simulink model "Main_SpeedOptimisedVersionTannenweg"  (R2024b)
settings: Solver=ode15s  StartTime=0.0  StopTime=3600*2  FixedStep=0.1  RelTol=0.001
model workspace (MAT data in the model file):
  Ti = 5
  fa = 0.00071
  fd = 0.03
  ips = 36
  ma = 0.0013
  md = 0.04
  roomarea1 = 20
  s = 15
libraries: fl_lib x1434, nesl_utility x105, SimscapeFluids_lib x35
(part 9 of 22)

== system Main_SpeedOptimisedVersionTannenweg/OG1/Raum3 ==
  Tatm : Inport
  valve command : Inport  Port=2
  Controlled Temperature Source : fl_lib/Thermal/Thermal Sources/Controlled Temperature Source
  Flur3EG : fl_lib/Thermal/Thermal Elements/Convective Heat Transfer  thermal_type=foundation.enum.constant_variable.constant  area=15.87 m^2  heat_tr_coeff=.8 W/m^2/K  min_heat_tr_coeff=1e-3 W/(K*m^2)  T_specify=off  T_priority=High  T=0 K  T_nominal_specify=off  T_nominal_value=1  T_nominal_unit=K  Q_specify=off  Q_priority=High  Q=0 J/s  Q_nominal_specify=off  Q_nominal_value=1  Q_nominal_unit=W
  Flur3OG2 : fl_lib/Thermal/Thermal Elements/Convective Heat Transfer  thermal_type=foundation.enum.constant_variable.constant  area=15.87 m^2  heat_tr_coeff=.8 W/m^2/K  min_heat_tr_coeff=1e-3 W/(K*m^2)  T_specify=off  T_priority=High  T=0 K  T_nominal_specify=off  T_nominal_value=1  T_nominal_unit=K  Q_specify=off  Q_priority=High  Q=0 J/s  Q_nominal_specify=off  Q_nominal_value=1  Q_nominal_unit=W
  Half Flur3EG : fl_lib/Thermal/Thermal Elements/Conductive Heat Transfer  thermal_type=foundation.enum.ConstantVariableTabulated.Constant  wall_geometry=foundation.enum.ConductionWallGeometry.Planar  area=15.87 m^2  thickness=.15 m  d_in=0.05 m  d_out=0.1 m  L=1 m  th_cond_min=10 W/(K*m)  th_cond=.32 W/m/K  th_cond_TLU=[413, 401, 392, 383, 371, 357, 342] W/(K*m)  temp_TLU=[200, 273, 400, 600, 800, 1000, 1200] K  T_specify=off  T_priority=High  T=0 K  T_nominal_specify=off  T_nominal_value=1  T_nominal_unit=K  Q_specify=off  Q_priority=High  Q=0 J/s  Q_nominal_specify=off  Q_nominal_value=1  Q_nominal_unit=W
  Half Flur3OG2 : fl_lib/Thermal/Thermal Elements/Conductive Heat Transfer  thermal_type=foundation.enum.ConstantVariableTabulated.Constant  wall_geometry=foundation.enum.ConductionWallGeometry.Planar  area=15.87 m^2  thickness=.15 m  d_in=0.05 m  d_out=0.1 m  L=1 m  th_cond_min=10 W/(K*m)  th_cond=.32 W/m/K  th_cond_TLU=[413, 401, 392, 383, 371, 357, 342] W/(K*m)  temp_TLU=[200, 273, 400, 600, 800, 1000, 1200] K  T_specify=off  T_priority=High  T=0 K  T_nominal_specify=off  T_nominal_value=1  T_nominal_unit=K  Q_specify=off  Q_priority=High  Q=0 J/s  Q_nominal_specify=off  Q_nominal_value=1  Q_nominal_unit=W
  Half IT-Air1 : fl_lib/Thermal/Thermal Elements/Conductive Heat Transfer  thermal_type=foundation.enum.ConstantVariableTabulated.Constant  wall_geometry=foundation.enum.ConductionWallGeometry.Planar  area=1.8 m^2  thickness=.022 m  d_in=0.05 m  d_out=0.1 m  L=1 m  th_cond_min=10 W/(K*m)  th_cond=.13 W/m/K  th_cond_TLU=[413, 401, 392, 383, 371, 357, 342] W/(K*m)  temp_TLU=[200, 273, 400, 600, 800, 1000, 1200] K  T_specify=off  T_priority=High  T=0 K  T_nominal_specify=off  T_nominal_value=1  T_nominal_unit=K  Q_specify=off  Q_priority=High  Q=0 J/s  Q_nominal_specify=off  Q_nominal_value=1  Q_nominal_unit=W
  Half IT-Air2 : fl_lib/Thermal/Thermal Elements/Conductive Heat Transfer  thermal_type=foundation.enum.ConstantVariableTabulated.Constant  wall_geometry=foundation.enum.ConductionWallGeometry.Planar  area=8.4 m^2  thickness=.022 m  d_in=0.05 m  d_out=0.1 m  L=1 m  th_cond_min=10 W/(K*m)  th_cond=.13 W/m/K  th_cond_TLU=[413, 401, 392, 383, 371, 357, 342] W/(K*m)  temp_TLU=[200, 273, 400, 600, 800, 1000, 1200] K  T_specify=off  T_priority=High  T=0 K  T_nominal_specify=off  T_nominal_value=1  T_nominal_unit=K  Q_specify=off  Q_priority=High  Q=0 J/s  Q_nominal_specify=off  Q_nominal_value=1  Q_nominal_unit=W
  Half IW1-Air : fl_lib/Thermal/Thermal Elements/Conductive Heat Transfer  thermal_type=foundation.enum.ConstantVariableTabulated.Constant  wall_geometry=foundation.enum.ConductionWallGeometry.Planar  area=6.7 m^2  thickness=.16 m  d_in=0.05 m  d_out=0.1 m  L=1 m  th_cond_min=10 W/(K*m)  th_cond=.069 W/m/K  th_cond_TLU=[413, 401, 392, 383, 371, 357, 342] W/(K*m)  temp_TLU=[200, 273, 400, 600, 800, 1000, 1200] K  T_specify=off  T_priority=High  T=0 K  T_nominal_specify=off  T_nominal_value=1  T_nominal_unit=K  Q_specify=off  Q_priority=High  Q=0 J/s  Q_nominal_specify=off  Q_nominal_value=1  Q_nominal_unit=W
  Half IW1-Air1 : fl_lib/Thermal/Thermal Elements/Conductive Heat Transfer  thermal_type=foundation.enum.ConstantVariableTabulated.Constant  wall_geometry=foundation.enum.ConductionWallGeometry.Planar  area=8.5 m^2  thickness=.16 m  d_in=0.05 m  d_out=0.1 m  L=1 m  th_cond_min=10 W/(K*m)  th_cond=.069 W/m/K  th_cond_TLU=[413, 401, 392, 383, 371, 357, 342] W/(K*m)  temp_TLU=[200, 273, 400, 600, 800, 1000, 1200] K  T_specify=off  T_priority=High  T=0 K  T_nominal_specify=off  T_nominal_value=1  T_nominal_unit=K  Q_specify=off  Q_priority=High  Q=0 J/s  Q_nominal_specify=off  Q_nominal_value=1  Q_nominal_unit=W
  Heater : Subsystem
      settings: PortSchema="{\"entries\":[{\"content\":{\"sides\":[{\"content\":{\"connectorIds\":[\"In1\"]},\"type\":\"ConnectorPlacement.EquallySpacedRectSide\",\"uuid\":\"7b4379d5-fe86-4f5f-b347-17463247d5cb\"},{\"content\":{\"connectorIds\":[\"RConn1\"],\"side\":\"RIGHT\"},\"type\":\"ConnectorPlacement.EquallySpacedRectSide\",\"uuid\":\"add3919f-9a79-4726-aacf-5344366c736f\"},{\"content\":{\"connectorIds\":[\"LConn1\"],\"side\":\"TOP\"},\"type\":\"ConnectorPlacement.EquallySpacedRectSide\",\"uuid\":\"2be7b118-9114-410d-904a-4756a3068fbb\"},{\"content\":{\"connectorIds\":[\"RConn2\"],\"side\":\"BOTTOM\"},\"type\":\"ConnectorPlacement.EquallySpacedRectSide\",\"uuid\":\"3477f1e1-5c09-4719-a7a1-17d4fd79a7ad\"}]},\"type\":\"ConnectorPlacement.EquallySpacedConnector\",\"uuid\":\"01d92670-8519-469a-8463-0c3952b88216\"}],\"packageUris\":[\"http://schema.mathworks.com/mf0/Connector/R2020b\"],\"version\":\"1.0\"}"
  IT3 : fl_lib/Thermal/Thermal Elements/Convective Heat Transfer  thermal_type=foundation.enum.constant_variable.constant  area=1.8 m^2  heat_tr_coeff=.8 W/m^2/K  min_heat_tr_coeff=1e-3 W/(K*m^2)  T_specify=off  T_priority=High  T=0 K  T_nominal_specify=off  T_nominal_value=1  T_nominal_unit=K  Q_specify=off  Q_priority=High  Q=0 J/s  Q_nominal_specify=off  Q_nominal_value=1  Q_nominal_unit=W
  IW3-12 : fl_lib/Thermal/Thermal Elements/Convective Heat Transfer  thermal_type=foundation.enum.constant_variable.constant  area=8.4 m^2  heat_tr_coeff=.8 W/m^2/K  min_heat_tr_coeff=1e-3 W/(K*m^2)  T_specify=off  T_priority=High  T=0 K  T_nominal_specify=off  T_nominal_value=1  T_nominal_unit=K  Q_specify=off  Q_priority=High  Q=0 J/s  Q_nominal_specify=off  Q_nominal_value=1  Q_nominal_unit=W
  IW3-2 : fl_lib/Thermal/Thermal Elements/Convective Heat Transfer  thermal_type=foundation.enum.constant_variable.constant  area=6.7 m^2  heat_tr_coeff=.8 W/m^2/K  min_heat_tr_coeff=1e-3 W/(K*m^2)  T_specify=off  T_priority=High  T=0 K  T_nominal_specify=off  T_nominal_value=1  T_nominal_unit=K  Q_specify=off  Q_priority=High  Q=0 J/s  Q_nominal_specify=off  Q_nominal_value=1  Q_nominal_unit=W
  IW3-4 : fl_lib/Thermal/Thermal Elements/Convective Heat Transfer  thermal_type=foundation.enum.constant_variable.constant  area=8.5 m^2  heat_tr_coeff=.8 W/m^2/K  min_heat_tr_coeff=1e-3 W/(K*m^2)  T_specify=off  T_priority=High  T=0 K  T_nominal_specify=off  T_nominal_value=1  T_nominal_unit=K  Q_specify=off  Q_priority=High  Q=0 J/s  Q_nominal_specify=off  Q_nominal_value=1  Q_nominal_unit=W
  Simulink-PS Converter3 : nesl_utility/Simulink-PS Converter  PhysicalDomain=network_engine_domain  SubClassName=ps_input  LeftPortType=input  RightPortType=output  PseudoPeriodic=off  Frequencies=[]  NoiseDistribution=none  NoiseParameters=[]  Unit=degC  AffineConversion=on  FilteringAndDerivatives=zero  SimscapeFilterOrder=1  InputFilterTimeConstant=.001  UdotUserProvided=0
  Temp. Sensor : Subsystem
  Thermal Mass 3-12 : fl_lib/Thermal/Thermal Elements/Thermal Mass  mass_type=foundation.enum.constant_variable.constant  mass=8.4*.15*547 kg  sp_heat=1600 J/kg/K  mass_min=1e-6 kg  num_ports=foundation.enum.numPorts2.one  m_specify=off  m_priority=High  m=1 kg  m_nominal_specify=off  m_nominal_value=1  m_nominal_unit=kg  T_specify=on  T_priority=High  T=Ti degC  T_nominal_specify=off  T_nominal_value=1  T_nominal_unit=K  Q_specify=off  Q_priority=None  Q=0 W  Q_nominal_specify=off  Q_nominal_value=1  Q_nominal_unit=W
  Thermal Mass Air : fl_lib/Thermal/Thermal Elements/Thermal Mass  mass_type=foundation.enum.constant_variable.constant  mass=48.7 kg  sp_heat=1005 J/kg/K  mass_min=1e-6 kg  num_ports=foundation.enum.numPorts2.one  m_specify=off  m_priority=High  m=1 kg  m_nominal_specify=off  m_nominal_value=1  m_nominal_unit=kg  T_specify=on  T_priority=High  T=Ti degC  T_nominal_specify=off  T_nominal_value=1  T_nominal_unit=K  Q_specify=off  Q_priority=None  Q=0 W  Q_nominal_specify=off  Q_nominal_value=1  Q_nominal_unit=W
  Thermal Mass Door3 : fl_lib/Thermal/Thermal Elements/Thermal Mass  mass_type=foundation.enum.constant_variable.constant  mass=36 kg  sp_heat=1600 J/kg/K  mass_min=1e-6 kg  num_ports=foundation.enum.numPorts2.one  m_specify=off  m_priority=High  m=1 kg  m_nominal_specify=off  m_nominal_value=1  m_nominal_unit=kg  T_specify=on  T_priority=High  T=Ti degC  T_nominal_specify=off  T_nominal_value=1  T_nominal_unit=K  Q_specify=off  Q_priority=None  Q=0 W  Q_nominal_specify=off  Q_nominal_value=1  Q_nominal_unit=W
  Thermal Mass Flur3EG : fl_lib/Thermal/Thermal Elements/Thermal Mass  mass_type=foundation.enum.constant_variable.constant  mass=4473 kg  sp_heat=889 J/kg/K  mass_min=1e-6 kg  num_ports=foundation.enum.numPorts2.one  m_specify=off  m_priority=High  m=1 kg  m_nominal_specify=off  m_nominal_value=1  m_nominal_unit=kg  T_specify=on  T_priority=High  T=Ti degC  T_nominal_specify=off  T_nominal_value=1  T_nominal_unit=K  Q_specify=off  Q_priority=None  Q=0 W  Q_nominal_specify=off  Q_nominal_value=1  Q_nominal_unit=W
  Thermal Mass Flur3OG2 : fl_lib/Thermal/Thermal Elements/Thermal Mass  mass_type=foundation.enum.constant_variable.constant  mass=4473 kg  sp_heat=889 J/kg/K  mass_min=1e-6 kg  num_ports=foundation.enum.numPorts2.one  m_specify=off  m_priority=High  m=1 kg  m_nominal_specify=off  m_nominal_value=1  m_nominal_unit=kg  T_specify=on  T_priority=High  T=Ti degC  T_nominal_specify=off  T_nominal_value=1  T_nominal_unit=K  Q_specify=off  Q_priority=None  Q=0 W  Q_nominal_specify=off  Q_nominal_value=1  Q_nominal_unit=W
  Thermal Mass IW3-2 : fl_lib/Thermal/Thermal Elements/Thermal Mass  mass_type=foundation.enum.constant_variable.constant  mass=6.7*.15*547 kg  sp_heat=1600 J/kg/K  mass_min=1e-6 kg  num_ports=foundation.enum.numPorts2.one  m_specify=off  m_priority=High  m=1 kg  m_nominal_specify=off  m_nominal_value=1  m_nominal_unit=kg  T_specify=on  T_priority=High  T=Ti degC  T_nominal_specify=off  T_nominal_value=1  T_nominal_unit=K  Q_specify=off  Q_priority=None  Q=0 W  Q_nominal_specify=off  Q_nominal_value=1  Q_nominal_unit=W
  Thermal Mass IW3-4 : fl_lib/Thermal/Thermal Elements/Thermal Mass  mass_type=foundation.enum.constant_variable.constant  mass=8.5*.15*547 kg  sp_heat=1600 J/kg/K  mass_min=1e-6 kg  num_ports=foundation.enum.numPorts2.one  m_specify=off  m_priority=High  m=1 kg  m_nominal_specify=off  m_nominal_value=1  m_nominal_unit=kg  T_specify=on  T_priority=High  T=Ti degC  T_nominal_specify=off  T_nominal_value=1  T_nominal_unit=K  Q_specify=off  Q_priority=None  Q=0 W  Q_nominal_specify=off  Q_nominal_value=1  Q_nominal_unit=W
  Thermal Reference1 : fl_lib/Thermal/Thermal Elements/Thermal Reference
  X-Atm : Subsystem
  Hot Water In1 : PMIOPort  Side=Left
  Y-Flur3OG2 : PMIOPort  Port=2  Side=Left
  Y-Flur3EG : PMIOPort  Port=3  Side=Left
  3-12 : PMIOPort  Port=4  Side=Left
  Door3 : PMIOPort  Port=5  Side=Left
  3-2 : PMIOPort  Port=6  Side=Right
  3-4 : PMIOPort  Port=7  Side=Right
  Hot Water Out1 : PMIOPort  Port=8  Side=Right
  Troom : Outport
  wires:
  Tatm/1 -> Simulink-PS Converter3/1
  Temp. Sensor/1(T) -> Troom/1
  valve command/1 -> Heater/1(valve command)
  connections:
  Flur3OG2/RConn1 -- Half Flur3OG2/LConn1
  Half Flur3OG2/RConn1 -- Y-Flur3OG2/RConn1 -- Thermal Mass Flur3OG2/LConn1
  IT3/RConn1 -- Half IT-Air1/LConn1
  Half IT-Air1/RConn1 -- Door3/RConn1 -- Thermal Mass Door3/LConn1
  IW3-12/RConn1 -- Half IT-Air2/LConn1
  3-12/RConn1 -- Thermal Mass 3-12/LConn1 -- Half IT-Air2/RConn1
  IW3-4/RConn1 -- Half IW1-Air1/LConn1
  3-4/RConn1 -- Half IW1-Air1/RConn1 -- Thermal Mass IW3-4/LConn1
  Heater/RConn2 -- Hot Water Out1/RConn1
  Hot Water In1/RConn1 -- Heater/LConn1
  X-Atm/RConn1 -- Controlled Temperature Source/LConn1
  Flur3EG/LConn1 -- Flur3OG2/LConn1 -- IW3-4/LConn1 -- Heater/RConn1 -- Thermal Mass Air/LConn1 -- X-Atm/LConn1 -- Temp. Sensor/LConn1 -- IW3-2/LConn1 -- IW3-12/LConn1 -- IT3/LConn1
  Controlled Temperature Source/RConn1 -- Simulink-PS Converter3/RConn1
  Thermal Reference1/LConn1 -- Controlled Temperature Source/RConn2
  Half IW1-Air/RConn1 -- Thermal Mass IW3-2/LConn1 -- 3-2/RConn1
  IW3-2/RConn1 -- Half IW1-Air/LConn1
  Half Flur3EG/RConn1 -- Thermal Mass Flur3EG/LConn1 -- Y-Flur3EG/RConn1
  Flur3EG/RConn1 -- Half Flur3EG/LConn1

== system Main_SpeedOptimisedVersionTannenweg/OG1/Raum4 ==
  valve command : Inport
  Tatm : Inport  Port=2
  Air-InnerDoor Convection1 : fl_lib/Thermal/Thermal Elements/Convective Heat Transfer  thermal_type=foundation.enum.constant_variable.constant  area=1.5 m^2  heat_tr_coeff=.8 W/m^2/K  min_heat_tr_coeff=1e-3 W/(K*m^2)  T_specify=off  T_priority=High  T=0 K  T_nominal_specify=off  T_nominal_value=1  T_nominal_unit=K  Q_specify=off  Q_priority=High  Q=0 J/s  Q_nominal_specify=off  Q_nominal_value=1  Q_nominal_unit=W
  Air-InnerWall IW4-1 : fl_lib/Thermal/Thermal Elements/Convective Heat Transfer  thermal_type=foundation.enum.constant_variable.constant  area=7.2 m^2  heat_tr_coeff=.8 W/m^2/K  min_heat_tr_coeff=1e-3 W/(K*m^2)  T_specify=off  T_priority=High  T=0 K  T_nominal_specify=off  T_nominal_value=1  T_nominal_unit=K  Q_specify=off  Q_priority=High  Q=0 J/s  Q_nominal_specify=off  Q_nominal_value=1  Q_nominal_unit=W
  Air-InnerWall IW4-2 : fl_lib/Thermal/Thermal Elements/Convective Heat Transfer  thermal_type=foundation.enum.constant_variable.constant  area=5.2 m^2  heat_tr_coeff=.8 W/m^2/K  min_heat_tr_coeff=1e-3 W/(K*m^2)  T_specify=off  T_priority=High  T=0 K  T_nominal_specify=off  T_nominal_value=1  T_nominal_unit=K  Q_specify=off  Q_priority=High  Q=0 J/s  Q_nominal_specify=off  Q_nominal_value=1  Q_nominal_unit=W
  Air-InnerWall IW4-3 : fl_lib/Thermal/Thermal Elements/Convective Heat Transfer  thermal_type=foundation.enum.constant_variable.constant  area=6.7 m^2  heat_tr_coeff=.8 W/m^2/K  min_heat_tr_coeff=1e-3 W/(K*m^2)  T_specify=off  T_priority=High  T=0 K  T_nominal_specify=off  T_nominal_value=1  T_nominal_unit=K  Q_specify=off  Q_priority=High  Q=0 J/s  Q_nominal_specify=off  Q_nominal_value=1  Q_nominal_unit=W
  Controlled Temperature Source : fl_lib/Thermal/Thermal Sources/Controlled Temperature Source
  Flur4EG : fl_lib/Thermal/Thermal Elements/Convective Heat Transfer  thermal_type=foundation.enum.constant_variable.constant  area=4.53 m^2  heat_tr_coeff=.8 W/m^2/K  min_heat_tr_coeff=1e-3 W/(K*m^2)  T_specify=off  T_priority=High  T=0 K  T_nominal_specify=off  T_nominal_value=1  T_nominal_unit=K  Q_specify=off  Q_priority=High  Q=0 J/s  Q_nominal_specify=off  Q_nominal_value=1  Q_nominal_unit=W
  Flur4OG2 : fl_lib/Thermal/Thermal Elements/Convective Heat Transfer  thermal_type=foundation.enum.constant_variable.constant  area=4.53 m^2  heat_tr_coeff=.8 W/m^2/K  min_heat_tr_coeff=1e-3 W/(K*m^2)  T_specify=off  T_priority=High  T=0 K  T_nominal_specify=off  T_nominal_value=1  T_nominal_unit=K  Q_specify=off  Q_priority=High  Q=0 J/s  Q_nominal_specify=off  Q_nominal_value=1  Q_nominal_unit=W
  Half Flur4EG : fl_lib/Thermal/Thermal Elements/Conductive Heat Transfer  thermal_type=foundation.enum.ConstantVariableTabulated.Constant  wall_geometry=foundation.enum.ConductionWallGeometry.Planar  area=4.53 m^2  thickness=.15 m  d_in=0.05 m  d_out=0.1 m  L=1 m  th_cond_min=10 W/(K*m)  th_cond=.32 W/m/K  th_cond_TLU=[413, 401, 392, 383, 371, 357, 342] W/(K*m)  temp_TLU=[200, 273, 400, 600, 800, 1000, 1200] K  T_specify=off  T_priority=High  T=0 K  T_nominal_specify=off  T_nominal_value=1  T_nominal_unit=K  Q_specify=off  Q_priority=High  Q=0 J/s  Q_nominal_specify=off  Q_nominal_value=1  Q_nominal_unit=W
  Half Flur4OG2 : fl_lib/Thermal/Thermal Elements/Conductive Heat Transfer  thermal_type=foundation.enum.ConstantVariableTabulated.Constant  wall_geometry=foundation.enum.ConductionWallGeometry.Planar  area=4.53 m^2  thickness=.15 m  d_in=0.05 m  d_out=0.1 m  L=1 m  th_cond_min=10 W/(K*m)  th_cond=.32 W/m/K  th_cond_TLU=[413, 401, 392, 383, 371, 357, 342] W/(K*m)  temp_TLU=[200, 273, 400, 600, 800, 1000, 1200] K  T_specify=off  T_priority=High  T=0 K  T_nominal_specify=off  T_nominal_value=1  T_nominal_unit=K  Q_specify=off  Q_priority=High  Q=0 J/s  Q_nominal_specify=off  Q_nominal_value=1  Q_nominal_unit=W
  Half Wall-Air Conduction1 : fl_lib/Thermal/Thermal Elements/Conductive Heat Transfer  thermal_type=foundation.enum.ConstantVariableTabulated.Constant  wall_geometry=foundation.enum.ConductionWallGeometry.Planar  area=7.2 m^2  thickness=.16 m  d_in=0.05 m  d_out=0.1 m  L=1 m  th_cond_min=10 W/(K*m)  th_cond=.069 W/m/K  th_cond_TLU=[413, 401, 392, 383, 371, 357, 342] W/(K*m)  temp_TLU=[200, 273, 400, 600, 800, 1000, 1200] K  T_specify=off  T_priority=High  T=0 K  T_nominal_specify=off  T_nominal_value=1  T_nominal_unit=K  Q_specify=off  Q_priority=High  Q=0 J/s  Q_nominal_specify=off  Q_nominal_value=1  Q_nominal_unit=W
  Half Wall-Air Conduction2 : fl_lib/Thermal/Thermal Elements/Conductive Heat Transfer  thermal_type=foundation.enum.ConstantVariableTabulated.Constant  wall_geometry=foundation.enum.ConductionWallGeometry.Planar  area=5.2 m^2  thickness=.16 m  d_in=0.05 m  d_out=0.1 m  L=1 m  th_cond_min=10 W/(K*m)  th_cond=.069 W/m/K  th_cond_TLU=[413, 401, 392, 383, 371, 357, 342] W/(K*m)  temp_TLU=[200, 273, 400, 600, 800, 1000, 1200] K  T_specify=off  T_priority=High  T=0 K  T_nominal_specify=off  T_nominal_value=1  T_nominal_unit=K  Q_specify=off  Q_priority=High  Q=0 J/s  Q_nominal_specify=off  Q_nominal_value=1  Q_nominal_unit=W
  Half Wall-Air Conduction3 : fl_lib/Thermal/Thermal Elements/Conductive Heat Transfer  thermal_type=foundation.enum.ConstantVariableTabulated.Constant  wall_geometry=foundation.enum.ConductionWallGeometry.Planar  area=6.7 m^2  thickness=.16 m  d_in=0.05 m  d_out=0.1 m  L=1 m  th_cond_min=10 W/(K*m)  th_cond=.069 W/m/K  th_cond_TLU=[413, 401, 392, 383, 371, 357, 342] W/(K*m)  temp_TLU=[200, 273, 400, 600, 800, 1000, 1200] K  T_specify=off  T_priority=High  T=0 K  T_nominal_specify=off  T_nominal_value=1  T_nominal_unit=K  Q_specify=off  Q_priority=High  Q=0 J/s  Q_nominal_specify=off  Q_nominal_value=1  Q_nominal_unit=W
  Half Window-Air Conduction1 : fl_lib/Thermal/Thermal Elements/Conductive Heat Transfer  thermal_type=foundation.enum.ConstantVariableTabulated.Constant  wall_geometry=foundation.enum.ConductionWallGeometry.Planar  area=1.5 m^2  thickness=.022 m  d_in=0.05 m  d_out=0.1 m  L=1 m  th_cond_min=10 W/(K*m)  th_cond=.13 W/m/K  th_cond_TLU=[413, 401, 392, 383, 371, 357, 342] W/(K*m)  temp_TLU=[200, 273, 400, 600, 800, 1000, 1200] K  T_specify=off  T_priority=High  T=0 K  T_nominal_specify=off  T_nominal_value=1  T_nominal_unit=K  Q_specify=off  Q_priority=High  Q=0 J/s  Q_nominal_specify=off  Q_nominal_value=1  Q_nominal_unit=W
  Heater : Subsystem
      settings: PortSchema="{\"entries\":[{\"content\":{\"sides\":[{\"content\":{\"connectorIds\":[\"In1\"]},\"type\":\"ConnectorPlacement.EquallySpacedRectSide\",\"uuid\":\"7b4379d5-fe86-4f5f-b347-17463247d5cb\"},{\"content\":{\"connectorIds\":[\"RConn1\"],\"side\":\"RIGHT\"},\"type\":\"ConnectorPlacement.EquallySpacedRectSide\",\"uuid\":\"add3919f-9a79-4726-aacf-5344366c736f\"},{\"content\":{\"connectorIds\":[\"LConn1\"],\"side\":\"TOP\"},\"type\":\"ConnectorPlacement.EquallySpacedRectSide\",\"uuid\":\"2be7b118-9114-410d-904a-4756a3068fbb\"},{\"content\":{\"connectorIds\":[\"RConn2\"],\"side\":\"BOTTOM\"},\"type\":\"ConnectorPlacement.EquallySpacedRectSide\",\"uuid\":\"3477f1e1-5c09-4719-a7a1-17d4fd79a7ad\"}]},\"type\":\"ConnectorPlacement.EquallySpacedConnector\",\"uuid\":\"01d92670-8519-469a-8463-0c3952b88216\"}],\"packageUris\":[\"http://schema.mathworks.com/mf0/Connector/R2020b\"],\"version\":\"1.0\"}"
  Simulink-PS Converter3 : nesl_utility/Simulink-PS Converter  PhysicalDomain=network_engine_domain  SubClassName=ps_input  LeftPortType=input  RightPortType=output  PseudoPeriodic=off  Frequencies=[]  NoiseDistribution=none  NoiseParameters=[]  Unit=degC  AffineConversion=on  FilteringAndDerivatives=zero  SimscapeFilterOrder=1  InputFilterTimeConstant=.001  UdotUserProvided=0
  Temp. Sensor : Subsystem
  Thermal Mass 4-1 : fl_lib/Thermal/Thermal Elements/Thermal Mass  mass_type=foundation.enum.constant_variable.constant  mass=7.2*.15*547 kg  sp_heat=876 J/kg/K  mass_min=1e-6 kg  num_ports=foundation.enum.numPorts2.one  m_specify=off  m_priority=High  m=1 kg  m_nominal_specify=off  m_nominal_value=1  m_nominal_unit=kg  T_specify=on  T_priority=High  T=Ti degC  T_nominal_specify=off  T_nominal_value=1  T_nominal_unit=K  Q_specify=off  Q_priority=None  Q=0 W  Q_nominal_specify=off  Q_nominal_value=1  Q_nominal_unit=W
  Thermal Mass 4-2 : fl_lib/Thermal/Thermal Elements/Thermal Mass  mass_type=foundation.enum.constant_variable.constant  mass=5.2*.15*547 kg  sp_heat=876 J/kg/K  mass_min=1e-6 kg  num_ports=foundation.enum.numPorts2.one  m_specify=off  m_priority=High  m=1 kg  m_nominal_specify=off  m_nominal_value=1  m_nominal_unit=kg  T_specify=on  T_priority=High  T=Ti degC  T_nominal_specify=off  T_nominal_value=1  T_nominal_unit=K  Q_specify=off  Q_priority=None  Q=0 W  Q_nominal_specify=off  Q_nominal_value=1  Q_nominal_unit=W
  Thermal Mass 4-3 : fl_lib/Thermal/Thermal Elements/Thermal Mass  mass_type=foundation.enum.constant_variable.constant  mass=6.7*.15*547 kg  sp_heat=876 J/kg/K  mass_min=1e-6 kg  num_ports=foundation.enum.numPorts2.one  m_specify=off  m_priority=High  m=1 kg  m_nominal_specify=off  m_nominal_value=1  m_nominal_unit=kg  T_specify=on  T_priority=High  T=Ti degC  T_nominal_specify=off  T_nominal_value=1  T_nominal_unit=K  Q_specify=off  Q_priority=None  Q=0 W  Q_nominal_specify=off  Q_nominal_value=1  Q_nominal_unit=W
  Thermal Mass Air : fl_lib/Thermal/Thermal Elements/Thermal Mass  mass_type=foundation.enum.constant_variable.constant  mass=13.9 kg  sp_heat=1005 J/kg/K  mass_min=1e-6 kg  num_ports=foundation.enum.numPorts2.one  m_specify=off  m_priority=High  m=1 kg  m_nominal_specify=off  m_nominal_value=1  m_nominal_unit=kg  T_specify=on  T_priority=High  T=Ti degC  T_nominal_specify=off  T_nominal_value=1  T_nominal_unit=K  Q_specify=off  Q_priority=None  Q=0 W  Q_nominal_specify=off  Q_nominal_value=1  Q_nominal_unit=W
  Thermal Mass Flur4EG : fl_lib/Thermal/Thermal Elements/Thermal Mass  mass_type=foundation.enum.constant_variable.constant  mass=1277 kg  sp_heat=889 J/kg/K  mass_min=1e-6 kg  num_ports=foundation.enum.numPorts2.one  m_specify=off  m_priority=High  m=1 kg  m_nominal_specify=off  m_nominal_value=1  m_nominal_unit=kg  T_specify=on  T_priority=High  T=Ti degC  T_nominal_specify=off  T_nominal_value=1  T_nominal_unit=K  Q_specify=off  Q_priority=None  Q=0 W  Q_nominal_specify=off  Q_nominal_value=1  Q_nominal_unit=W
  Thermal Mass Flur4OG2 : fl_lib/Thermal/Thermal Elements/Thermal Mass  mass_type=foundation.enum.constant_variable.constant  mass=1277 kg  sp_heat=889 J/kg/K  mass_min=1e-6 kg  num_ports=foundation.enum.numPorts2.one  m_specify=off  m_priority=High  m=1 kg  m_nominal_specify=off  m_nominal_value=1  m_nominal_unit=kg  T_specify=on  T_priority=High  T=Ti degC  T_nominal_specify=off  T_nominal_value=1  T_nominal_unit=K  Q_specify=off  Q_priority=None  Q=0 W  Q_nominal_specify=off  Q_nominal_value=1  Q_nominal_unit=W
  Thermal Mass InnerDoor : fl_lib/Thermal/Thermal Elements/Thermal Mass  mass_type=foundation.enum.constant_variable.constant  mass=30 kg  sp_heat=1600 J/kg/K  mass_min=1e-6 kg  num_ports=foundation.enum.numPorts2.one  m_specify=off  m_priority=High  m=1 kg  m_nominal_specify=off  m_nominal_value=1  m_nominal_unit=kg  T_specify=on  T_priority=High  T=Ti degC  T_nominal_specify=off  T_nominal_value=1  T_nominal_unit=K  Q_specify=off  Q_priority=None  Q=0 W  Q_nominal_specify=off  Q_nominal_value=1  Q_nominal_unit=W
  Thermal Reference1 : fl_lib/Thermal/Thermal Elements/Thermal Reference
  X-Atm : Subsystem
  Hot Water In1 : PMIOPort  Side=Left
  4-3 : PMIOPort  Port=2  Side=Left
  Door4 : PMIOPort  Port=3  Side=Left
  4-2 : PMIOPort  Port=4  Side=Left
  4-1 : PMIOPort  Port=5  Side=Left
  Y-Flur4OG2 : PMIOPort  Port=6  Side=Right
  Y-Flur4EG : PMIOPort  Port=7  Side=Right
  Hot Water Out1 : PMIOPort  Port=8  Side=Right
  Troom : Outport
  wires:
  Tatm/1 -> Simulink-PS Converter3/1
  Temp. Sensor/1(T) -> Troom/1
  valve command/1 -> Heater/1(valve command)
  connections:
  Flur4OG2/RConn1 -- Half Flur4OG2/LConn1
  Half Flur4OG2/RConn1 -- Y-Flur4OG2/RConn1 -- Thermal Mass Flur4OG2/LConn1
  Air-InnerWall IW4-3/RConn1 -- Half Wall-Air Conduction3/LConn1
  Air-InnerWall IW4-2/RConn1 -- Half Wall-Air Conduction2/LConn1
  Air-InnerWall IW4-1/RConn1 -- Half Wall-Air Conduction1/LConn1
  Air-InnerDoor Convection1/RConn1 -- Half Window-Air Conduction1/LConn1
  Thermal Mass 4-3/LConn1 -- 4-3/RConn1 -- Half Wall-Air Conduction3/RConn1
  Door4/RConn1 -- Half Window-Air Conduction1/RConn1 -- Thermal Mass InnerDoor/LConn1
  4-1/RConn1 -- Half Wall-Air Conduction1/RConn1 -- Thermal Mass 4-1/LConn1
  Half Wall-Air Conduction2/RConn1 -- 4-2/RConn1 -- Thermal Mass 4-2/LConn1
  Heater/RConn2 -- Hot Water Out1/RConn1
  Hot Water In1/RConn1 -- Heater/LConn1
  X-Atm/RConn1 -- Controlled Temperature Source/LConn1
  Controlled Temperature Source/RConn1 -- Simulink-PS Converter3/RConn1
  Thermal Reference1/LConn1 -- Controlled Temperature Source/RConn2
  Half Flur4EG/RConn1 -- Thermal Mass Flur4EG/LConn1 -- Y-Flur4EG/RConn1
  Flur4EG/RConn1 -- Half Flur4EG/LConn1
  Flur4EG/LConn1 -- Air-InnerWall IW4-3/LConn1 -- Air-InnerWall IW4-2/LConn1 -- Air-InnerWall IW4-1/LConn1 -- Heater/RConn1 -- Thermal Mass Air/LConn1 -- X-Atm/LConn1 -- Temp. Sensor/LConn1 -- Air-InnerDoor Convection1/LConn1 -- Flur4OG2/LConn1

== system Main_SpeedOptimisedVersionTannenweg/OG1/Raum5 ==
  Tatm : Inport
  valve command : Inport  Port=2
  Air-InnerDoor Convection1 : fl_lib/Thermal/Thermal Elements/Convective Heat Transfer  thermal_type=foundation.enum.constant_variable.constant  area=1.8 m^2  heat_tr_coeff=.8 W/m^2/K  min_heat_tr_coeff=1e-3 W/(K*m^2)  T_specify=off  T_priority=High  T=0 K  T_nominal_specify=off  T_nominal_value=1  T_nominal_unit=K  Q_specify=off  Q_priority=High  Q=0 J/s  Q_nominal_specify=off  Q_nominal_value=1  Q_nominal_unit=W
  Air-InnerWall 5-9 : fl_lib/Thermal/Thermal Elements/Convective Heat Transfer  thermal_type=foundation.enum.constant_variable.constant  area=9.3 m^2  heat_tr_coeff=.8 W/m^2/K  min_heat_tr_coeff=1e-3 W/(K*m^2)  T_specify=off  T_priority=High  T=0 K  T_nominal_specify=off  T_nominal_value=1  T_nominal_unit=K  Q_specify=off  Q_priority=High  Q=0 J/s  Q_nominal_specify=off  Q_nominal_value=1  Q_nominal_unit=W
  Controlled Temperature Source : fl_lib/Thermal/Thermal Sources/Controlled Temperature Source
  Flur5EG : fl_lib/Thermal/Thermal Elements/Convective Heat Transfer  thermal_type=foundation.enum.constant_variable.constant  area=13.58 m^2  heat_tr_coeff=.8 W/m^2/K  min_heat_tr_coeff=1e-3 W/(K*m^2)  T_specify=off  T_priority=High  T=0 K  T_nominal_specify=off  T_nominal_value=1  T_nominal_unit=K  Q_specify=off  Q_priority=High  Q=0 J/s  Q_nominal_specify=off  Q_nominal_value=1  Q_nominal_unit=W
  Flur5OG2 : fl_lib/Thermal/Thermal Elements/Convective Heat Transfer  thermal_type=foundation.enum.constant_variable.constant  area=13.58 m^2  heat_tr_coeff=.8 W/m^2/K  min_heat_tr_coeff=1e-3 W/(K*m^2)  T_specify=off  T_priority=High  T=0 K  T_nominal_specify=off  T_nominal_value=1  T_nominal_unit=K  Q_specify=off  Q_priority=High  Q=0 J/s  Q_nominal_specify=off  Q_nominal_value=1  Q_nominal_unit=W
  Half Flur5EG : fl_lib/Thermal/Thermal Elements/Conductive Heat Transfer  thermal_type=foundation.enum.ConstantVariableTabulated.Constant  wall_geometry=foundation.enum.ConductionWallGeometry.Planar  area=13.58 m^2  thickness=.15 m  d_in=0.05 m  d_out=0.1 m  L=1 m  th_cond_min=10 W/(K*m)  th_cond=.32 W/m/K  th_cond_TLU=[413, 401, 392, 383, 371, 357, 342] W/(K*m)  temp_TLU=[200, 273, 400, 600, 800, 1000, 1200] K  T_specify=off  T_priority=High  T=0 K  T_nominal_specify=off  T_nominal_value=1  T_nominal_unit=K  Q_specify=off  Q_priority=High  Q=0 J/s  Q_nominal_specify=off  Q_nominal_value=1  Q_nominal_unit=W
  Half Flur5OG2 : fl_lib/Thermal/Thermal Elements/Conductive Heat Transfer  thermal_type=foundation.enum.ConstantVariableTabulated.Constant  wall_geometry=foundation.enum.ConductionWallGeometry.Planar  area=13.58 m^2  thickness=.15 m  d_in=0.05 m  d_out=0.1 m  L=1 m  th_cond_min=10 W/(K*m)  th_cond=.32 W/m/K  th_cond_TLU=[413, 401, 392, 383, 371, 357, 342] W/(K*m)  temp_TLU=[200, 273, 400, 600, 800, 1000, 1200] K  T_specify=off  T_priority=High  T=0 K  T_nominal_specify=off  T_nominal_value=1  T_nominal_unit=K  Q_specify=off  Q_priority=High  Q=0 J/s  Q_nominal_specify=off  Q_nominal_value=1  Q_nominal_unit=W
  Half Wall-Air Conduction1 : fl_lib/Thermal/Thermal Elements/Conductive Heat Transfer  thermal_type=foundation.enum.ConstantVariableTabulated.Constant  wall_geometry=foundation.enum.ConductionWallGeometry.Planar  area=9.3 m^2  thickness=.16 m  d_in=0.05 m  d_out=0.1 m  L=1 m  th_cond_min=10 W/(K*m)  th_cond=.069 W/m/K  th_cond_TLU=[413, 401, 392, 383, 371, 357, 342] W/(K*m)  temp_TLU=[200, 273, 400, 600, 800, 1000, 1200] K  T_specify=off  T_priority=High  T=0 K  T_nominal_specify=off  T_nominal_value=1  T_nominal_unit=K  Q_specify=off  Q_priority=High  Q=0 J/s  Q_nominal_specify=off  Q_nominal_value=1  Q_nominal_unit=W
  Half Wall-Air Conduction2 : fl_lib/Thermal/Thermal Elements/Conductive Heat Transfer  thermal_type=foundation.enum.ConstantVariableTabulated.Constant  wall_geometry=foundation.enum.ConductionWallGeometry.Planar  area=2.5 m^2  thickness=.16 m  d_in=0.05 m  d_out=0.1 m  L=1 m  th_cond_min=10 W/(K*m)  th_cond=.069 W/m/K  th_cond_TLU=[413, 401, 392, 383, 371, 357, 342] W/(K*m)  temp_TLU=[200, 273, 400, 600, 800, 1000, 1200] K  T_specify=off  T_priority=High  T=0 K  T_nominal_specify=off  T_nominal_value=1  T_nominal_unit=K  Q_specify=off  Q_priority=High  Q=0 J/s  Q_nominal_specify=off  Q_nominal_value=1  Q_nominal_unit=W
  Half Wall-Air Conduction3 : fl_lib/Thermal/Thermal Elements/Conductive Heat Transfer  thermal_type=foundation.enum.ConstantVariableTabulated.Constant  wall_geometry=foundation.enum.ConductionWallGeometry.Planar  area=9.3 m^2  thickness=.16 m  d_in=0.05 m  d_out=0.1 m  L=1 m  th_cond_min=10 W/(K*m)  th_cond=.069 W/m/K  th_cond_TLU=[413, 401, 392, 383, 371, 357, 342] W/(K*m)  temp_TLU=[200, 273, 400, 600, 800, 1000, 1200] K  T_specify=off  T_priority=High  T=0 K  T_nominal_specify=off  T_nominal_value=1  T_nominal_unit=K  Q_specify=off  Q_priority=High  Q=0 J/s  Q_nominal_specify=off  Q_nominal_value=1  Q_nominal_unit=W
  Half Window-Air Conduction1 : fl_lib/Thermal/Thermal Elements/Conductive Heat Transfer  thermal_type=foundation.enum.ConstantVariableTabulated.Constant  wall_geometry=foundation.enum.ConductionWallGeometry.Planar  area=1.8 m^2  thickness=.022 m  d_in=0.05 m  d_out=0.1 m  L=1 m  th_cond_min=10 W/(K*m)  th_cond=.13 W/m/K  th_cond_TLU=[413, 401, 392, 383, 371, 357, 342] W/(K*m)  temp_TLU=[200, 273, 400, 600, 800, 1000, 1200] K  T_specify=off  T_priority=High  T=0 K  T_nominal_specify=off  T_nominal_value=1  T_nominal_unit=K  Q_specify=off  Q_priority=High  Q=0 J/s  Q_nominal_specify=off  Q_nominal_value=1  Q_nominal_unit=W
  Heater : Subsystem
      settings: PortSchema="{\"entries\":[{\"content\":{\"sides\":[{\"content\":{\"connectorIds\":[\"In1\"]},\"type\":\"ConnectorPlacement.EquallySpacedRectSide\",\"uuid\":\"7b4379d5-fe86-4f5f-b347-17463247d5cb\"},{\"content\":{\"connectorIds\":[\"RConn1\"],\"side\":\"RIGHT\"},\"type\":\"ConnectorPlacement.EquallySpacedRectSide\",\"uuid\":\"add3919f-9a79-4726-aacf-5344366c736f\"},{\"content\":{\"connectorIds\":[\"LConn1\"],\"side\":\"TOP\"},\"type\":\"ConnectorPlacement.EquallySpacedRectSide\",\"uuid\":\"2be7b118-9114-410d-904a-4756a3068fbb\"},{\"content\":{\"connectorIds\":[\"RConn2\"],\"side\":\"BOTTOM\"},\"type\":\"ConnectorPlacement.EquallySpacedRectSide\",\"uuid\":\"3477f1e1-5c09-4719-a7a1-17d4fd79a7ad\"}]},\"type\":\"ConnectorPlacement.EquallySpacedConnector\",\"uuid\":\"01d92670-8519-469a-8463-0c3952b88216\"}],\"packageUris\":[\"http://schema.mathworks.com/mf0/Connector/R2020b\"],\"version\":\"1.0\"}"
  IW5-6 : fl_lib/Thermal/Thermal Elements/Convective Heat Transfer  thermal_type=foundation.enum.constant_variable.constant  area=9.3 m^2  heat_tr_coeff=.8 W/m^2/K  min_heat_tr_coeff=1e-3 W/(K*m^2)  T_specify=off  T_priority=High  T=0 K  T_nominal_specify=off  T_nominal_value=1  T_nominal_unit=K  Q_specify=off  Q_priority=High  Q=0 J/s  Q_nominal_specify=off  Q_nominal_value=1  Q_nominal_unit=W
  IW5-7 : fl_lib/Thermal/Thermal Elements/Convective Heat Transfer  thermal_type=foundation.enum.constant_variable.constant  area=2.5 m^2  heat_tr_coeff=.8 W/m^2/K  min_heat_tr_coeff=1e-3 W/(K*m^2)  T_specify=off  T_priority=High  T=0 K  T_nominal_specify=off  T_nominal_value=1  T_nominal_unit=K  Q_specify=off  Q_priority=High  Q=0 J/s  Q_nominal_specify=off  Q_nominal_value=1  Q_nominal_unit=W
  Simulink-PS Converter3 : nesl_utility/Simulink-PS Converter  PhysicalDomain=network_engine_domain  SubClassName=ps_input  LeftPortType=input  RightPortType=output  PseudoPeriodic=off  Frequencies=[]  NoiseDistribution=none  NoiseParameters=[]  Unit=degC  AffineConversion=on  FilteringAndDerivatives=zero  SimscapeFilterOrder=1  InputFilterTimeConstant=.001  UdotUserProvided=0
  Temp. Sensor : Subsystem
  Thermal Mass 5-6 : fl_lib/Thermal/Thermal Elements/Thermal Mass  mass_type=foundation.enum.constant_variable.constant  mass=9.3*.15*547 kg  sp_heat=876 J/kg/K  mass_min=1e-6 kg  num_ports=foundation.enum.numPorts2.one  m_specify=off  m_priority=High  m=1 kg  m_nominal_specify=off  m_nominal_value=1  m_nominal_unit=kg  T_specify=on  T_priority=High  T=Ti degC  T_nominal_specify=off  T_nominal_value=1  T_nominal_unit=K  Q_specify=off  Q_priority=None  Q=0 W  Q_nominal_specify=off  Q_nominal_value=1  Q_nominal_unit=W
  Thermal Mass 5-7 : fl_lib/Thermal/Thermal Elements/Thermal Mass  mass_type=foundation.enum.constant_variable.constant  mass=2.5*.15*547 kg  sp_heat=876 J/kg/K  mass_min=1e-6 kg  num_ports=foundation.enum.numPorts2.one  m_specify=off  m_priority=High  m=1 kg  m_nominal_specify=off  m_nominal_value=1  m_nominal_unit=kg  T_specify=on  T_priority=High  T=Ti degC  T_nominal_specify=off  T_nominal_value=1  T_nominal_unit=K  Q_specify=off  Q_priority=None  Q=0 W  Q_nominal_specify=off  Q_nominal_value=1  Q_nominal_unit=W
  Thermal Mass 5-9 : fl_lib/Thermal/Thermal Elements/Thermal Mass  mass_type=foundation.enum.constant_variable.constant  mass=9.3*.15*547 kg  sp_heat=876 J/kg/K  mass_min=1e-6 kg  num_ports=foundation.enum.numPorts2.one  m_specify=off  m_priority=High  m=1 kg  m_nominal_specify=off  m_nominal_value=1  m_nominal_unit=kg  T_specify=on  T_priority=High  T=Ti degC  T_nominal_specify=off  T_nominal_value=1  T_nominal_unit=K  Q_specify=off  Q_priority=None  Q=0 W  Q_nominal_specify=off  Q_nominal_value=1  Q_nominal_unit=W
  Thermal Mass Air : fl_lib/Thermal/Thermal Elements/Thermal Mass  mass_type=foundation.enum.constant_variable.constant  mass=48.7 kg  sp_heat=1005 J/kg/K  mass_min=1e-6 kg  num_ports=foundation.enum.numPorts2.one  m_specify=off  m_priority=High  m=1 kg  m_nominal_specify=off  m_nominal_value=1  m_nominal_unit=kg  T_specify=on  T_priority=High  T=Ti degC  T_nominal_specify=off  T_nominal_value=1  T_nominal_unit=K  Q_specify=off  Q_priority=None  Q=0 W  Q_nominal_specify=off  Q_nominal_value=1  Q_nominal_unit=W
  Thermal Mass Flur5EG : fl_lib/Thermal/Thermal Elements/Thermal Mass  mass_type=foundation.enum.constant_variable.constant  mass=3828 kg  sp_heat=889 J/kg/K  mass_min=1e-6 kg  num_ports=foundation.enum.numPorts2.one  m_specify=off  m_priority=High  m=1 kg  m_nominal_specify=off  m_nominal_value=1  m_nominal_unit=kg  T_specify=on  T_priority=High  T=Ti degC  T_nominal_specify=off  T_nominal_value=1  T_nominal_unit=K  Q_specify=off  Q_priority=None  Q=0 W  Q_nominal_specify=off  Q_nominal_value=1  Q_nominal_unit=W
  Thermal Mass Flur5OG2 : fl_lib/Thermal/Thermal Elements/Thermal Mass  mass_type=foundation.enum.constant_variable.constant  mass=3828 kg  sp_heat=889 J/kg/K  mass_min=1e-6 kg  num_ports=foundation.enum.numPorts2.one  m_specify=off  m_priority=High  m=1 kg  m_nominal_specify=off  m_nominal_value=1  m_nominal_unit=kg  T_specify=on  T_priority=High  T=Ti degC  T_nominal_specify=off  T_nominal_value=1  T_nominal_unit=K  Q_specify=off  Q_priority=None  Q=0 W  Q_nominal_specify=off  Q_nominal_value=1  Q_nominal_unit=W
  Thermal Mass InnerDoor : fl_lib/Thermal/Thermal Elements/Thermal Mass  mass_type=foundation.enum.constant_variable.constant  mass=36 kg  sp_heat=1600 J/kg/K  mass_min=1e-6 kg  num_ports=foundation.enum.numPorts2.one  m_specify=off  m_priority=High  m=1 kg  m_nominal_specify=off  m_nominal_value=1  m_nominal_unit=kg  T_specify=on  T_priority=High  T=Ti degC  T_nominal_specify=off  T_nominal_value=1  T_nominal_unit=K  Q_specify=off  Q_priority=None  Q=0 W  Q_nominal_specify=off  Q_nominal_value=1  Q_nominal_unit=W
  Thermal Reference1 : fl_lib/Thermal/Thermal Elements/Thermal Reference
  X-Atm : Subsystem
  Door5 : PMIOPort  Side=Left
  5-7 : PMIOPort  Port=2  Side=Left
  Hot Water In1 : PMIOPort  Port=3  Side=Left
  5-9 : PMIOPort  Port=4  Side=Left
  Y-Flur5EG : PMIOPort  Port=5  Side=Right
  Y-Flur5OG2 : PMIOPort  Port=6  Side=Right
  Hot Water Out1 : PMIOPort  Port=7  Side=Right
  5-6 : PMIOPort  Port=8  Side=Right
  Troom : Outport
  wires:
  Temp. Sensor/1(T) -> Troom/1
  Tatm/1 -> Simulink-PS Converter3/1
  valve command/1 -> Heater/1(valve command)
  connections:
  Flur5OG2/RConn1 -- Half Flur5OG2/LConn1
  Half Flur5OG2/RConn1 -- Y-Flur5OG2/RConn1 -- Thermal Mass Flur5OG2/LConn1
  IW5-7/RConn1 -- Half Wall-Air Conduction2/LConn1
  IW5-6/RConn1 -- Half Wall-Air Conduction1/LConn1
  Air-InnerDoor Convection1/RConn1 -- Half Window-Air Conduction1/LConn1
  Air-InnerWall 5-9/RConn1 -- Half Wall-Air Conduction3/LConn1
  Half Window-Air Conduction1/RConn1 -- Door5/RConn1 -- Thermal Mass InnerDoor/LConn1
  Thermal Mass 5-9/LConn1 -- 5-9/RConn1 -- Half Wall-Air Conduction3/RConn1
  5-7/RConn1 -- Thermal Mass 5-7/LConn1 -- Half Wall-Air Conduction2/RConn1
  Thermal Mass 5-6/LConn1 -- 5-6/RConn1 -- Half Wall-Air Conduction1/RConn1
  Flur5OG2/LConn1 -- Air-InnerWall 5-9/LConn1 -- IW5-7/LConn1 -- IW5-6/LConn1 -- Heater/RConn1 -- Thermal Mass Air/LConn1 -- Temp. Sensor/LConn1 -- X-Atm/LConn1 -- Air-InnerDoor Convection1/LConn1 -- Flur5EG/LConn1
  Thermal Reference1/LConn1 -- Controlled Temperature Source/RConn2
  Controlled Temperature Source/RConn1 -- Simulink-PS Converter3/RConn1
  X-Atm/RConn1 -- Controlled Temperature Source/LConn1
  Hot Water In1/RConn1 -- Heater/LConn1
  Heater/RConn2 -- Hot Water Out1/RConn1
  Half Flur5EG/RConn1 -- Thermal Mass Flur5EG/LConn1 -- Y-Flur5EG/RConn1
  Flur5EG/RConn1 -- Half Flur5EG/LConn1
